simulink model "FMT_GroundRHS"  (R2026b)
settings: Solver=FixedStepDiscrete  StopTime=2  FixedStep=0.0005
settings Model: DataDictionary=Flight_Parameters.sldd  Creator=26718  LastModifiedBy=26718

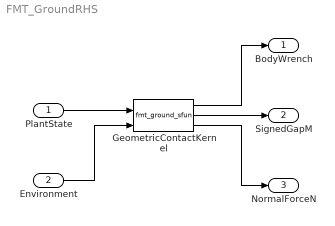
== system FMT_GroundRHS ==
  PlantState : Inport  OutDataTypeStr=double  PortDimensions=17
  Environment : Inport  Port=2  OutDataTypeStr=double  PortDimensions=15
  GeometricContactKernel : S-Function  FunctionName=fmt_ground_sfun  Parameters=PlantParameters  SFunctionDeploymentMode=off  EnableBusSupport=off
  BodyWrench : Outport
  SignedGapM : Outport  Port=2
  NormalForceN : Outport  Port=3
  wires:
  GeometricContactKernel/3 -> NormalForceN/1
  GeometricContactKernel/2 -> SignedGapM/1
  Environment/1 -> GeometricContactKernel/2
  PlantState/1 -> GeometricContactKernel/1
  GeometricContactKernel/1 -> BodyWrench/1
